simulink model "ftc_biodiesel"  (R2026b)
settings: Solver=ode15s  StopTime=120  MaxStep=0.25  RelTol=1e-7  AbsTol=1e-9
InitFcn:
  | ftc_supervisor('init', sup_cfg);
values from neighbouring files (symbols this model uses):
  P = rmfield(P, 'names')    [build_ftc_sim.m]    (also in ftc_check.m = ftc_params(); ftc_supervisor.m = S.P)
undefined symbols (not defined in the file or in its folder): ctrl_mode, t_f
libraries: slpidlib x1
settings Model: Creator=Joseph  LastModifiedBy=Joseph

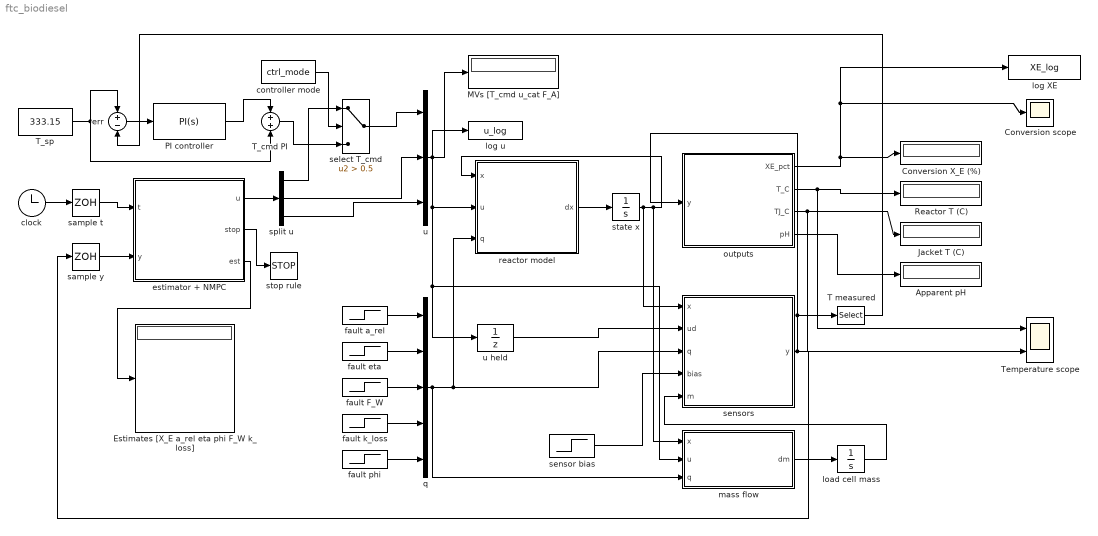
== system ftc_biodiesel ==
  Apparent pH : Display
  Conversion X_E (%) : Display
  Conversion scope : Scope
  Estimates [X_E a_rel eta phi F_W k_loss] : Display
  Jacket T (C) : Display
  MVs [T_cmd u_cat F_A] : Display
  PI controller : slpidlib/PID Controller  Controller=PI  Form=Parallel  TimeDomain=Continuous-time  UseExternalTs=off  SampleTime=-1  IntegratorMethod=Forward Euler  FilterMethod=Forward Euler  ControllerParametersSource=internal  P=6  I=6/8  UseKiTs=off  D=0  UseExternalDerivativeSource=off  N=100  UseFilter=on  TunerSelectOption=Transfer Function Based (PID Tuner App)  InitialConditionSource=internal  InitialConditionForIntegrator=0  InitialConditionForFilter=0  DifferentiatorICPrevScaledInput=0  ExternalReset=none  TrackingMode=off  Kt=1  LimitOutput=on  SatLimitsSource=internal  UpperSaturationLimit=353.15-333.15  LowerSaturationLimit=298.15-333.15  LinearizeAsGain=on  AntiWindupMode=back-calculation  Kb=1/8  LimitIntegrator=off  UpperIntegratorSaturationLimit=inf  LowerIntegratorSaturationLimit=-inf  POutMin=[]  POutMax=[]  IOutMin=[]  IOutMax=[]  DOutMin=[]  DOutMax=[]  NOutMin=[]  NOutMax=[]  SumOutMin=[]  SumOutMax=[]  SaturationOutMin=[]  SaturationOutMax=[]  PParamMin=[]  PParamMax=[]  IParamMin=[]  IParamMax=[]  DParamMin=[]  DParamMax=[]  NParamMin=[]  NParamMax=[]  KbParamMin=[]  KbParamMax=[]  KtParamMin=[]  KtParamMax=[]  KbOutMin=[]  KbOutMax=[]  KtOutMin=[]  KtOutMax=[]  IntegratorOutMin=[]  IntegratorOutMax=[]  FilterOutMin=[]  FilterOutMax=[]  SumI1OutMin=[]  SumI1OutMax=[]  SumI2OutMin=[]  SumI2OutMax=[]  SumI3OutMin=[]  SumI3OutMax=[]  SumI4OutMin=[]  SumI4OutMax=[]  SumDOutMin=[]  SumDOutMax=[]  DifferentiatorOutMin=[]  DifferentiatorOutMax=[]  FilterDiffOutCoefMin=[]  FilterDiffOutCoefMax=[]  ReciprocalOutMin=[]  ReciprocalOutMax=[]  SumDenOutMin=[]  SumDenOutMax=[]  SumNumOutMin=[]  SumNumOutMax=[]  DivideOutMin=[]  DivideOutMax=[]  UdiffTsProdOutMin=[]  UdiffTsProdOutMax=[]  NTsProdOutMin=[]  NTsProdOutMax=[]  UintegralTsProdOutMin=[]  UintegralTsProdOutMax=[]  UngainTsProdOutMin=[]  UngainTsProdOutMax=[]  ClampingZeroOutDataTypeStr=Inherit: Inherit via back propagation  ClampingZeroOutMin=[]  ClampingZeroOutMax=[]  FilterDenConstantOutDataTypeStr=Inherit: Inherit via back propagation  FilterDenConstantOutMin=[]  FilterDenConstantOutMax=[]  PCopyOutDataTypeStr=Inherit: Inherit via back propagation  PCopyOutMin=[]  PCopyOutMax=[]  NCopyOutDataTypeStr=Inherit: Inherit via back propagation  NCopyOutMin=[]  NCopyOutMax=[]  IntegratorContinuousStateAttributes=''  IntegratorStateMustResolveToSignalObject=off  IntegratorRTWStateStorageClass=Auto  FilterContinuousStateAttributes=''  FilterStateMustResolveToSignalObject=off  FilterRTWStateStorageClass=Auto  ParallelPVariant=InternalParameters  IdealPVariant=Disabled  IVariant=InternalParameters  DVariant=Disabled  IntegratorVariant=Continuous  SatVariant=Enabled  AWVariant=BackCalculation  PCopyVariant=Disabled  TRVariant=Disabled  FdbkBlocksVariant=Forward  IdealPFdbkVariant=Disabled  SatFdbkVariant=Disabled  DerivativeFilterVariant=Disabled  NVariant=Disabled  NCopyVariant=Disabled_SignalSpec  FilterICVariant=Disabled  IntegratorICVariant=InternalICs  ExternalResetVariant=Disabled  TRSumVariant=Passthrough  SumFdbkVariant=Disabled  SumVariant=Sum_PI  TsampFilterVariant=InternalTs  TsampNgainVariant=Passthrough  TsampIntegralVariant=Disabled_SignalSpec  ExternalSaturationOutDataTypeStr=Inherit: Same as second input  DerivativeSourceVariant=Disabled  PreIntVariant=InternalPreInt
  Reactor T (C) : Display
  T measured : Selector  InputPortWidth=9  IndexOptions=Index vector (dialog)  Indices=1  OutputSizes=1
  T_cmd PI : Sum
  T_sp : Constant  Value=333.15
  Temperature scope : Scope  NumInputPorts=2
  clock : Clock
  controller mode : Constant  Value=ctrl_mode
  err : Sum  Inputs=+-
  estimator + NMPC : MATLAB Function  TreatAsAtomicUnit=on
  fault F_W : Step  Time=t_f  FinalValue=FW_f  SampleTime=0
  fault a_rel : Step  Time=t_f  InitialValue=1  FinalValue=a_f  SampleTime=0
  fault eta : Step  Time=t_f  InitialValue=1  FinalValue=eta_f  SampleTime=0
  fault k_loss : Step  Time=t_f  FinalValue=kl_f  SampleTime=0
  fault phi : Step  Time=t_f  InitialValue=1  FinalValue=phi_f  SampleTime=0
  load cell mass : Integrator
  log XE : ToWorkspace  VariableName=XE_log  SaveFormat=Timeseries  SampleTime=-1
  log u : ToWorkspace  VariableName=u_log  SaveFormat=Timeseries  SampleTime=-1
  mass flow : MATLAB Function  TreatAsAtomicUnit=on
  outputs : MATLAB Function  TreatAsAtomicUnit=on
  q : Mux  Inputs=5
  reactor model : MATLAB Function  TreatAsAtomicUnit=on
  sample t : ZeroOrderHold  SampleTime=0.25
  sample y : ZeroOrderHold  SampleTime=0.25
  select T_cmd : Switch  Criteria=u2 > Threshold  Threshold=0.5  SaturateOnIntegerOverflow=off  InputSameDT=off
  sensor bias : Step  Time=t_f  FinalValue=bias_f  SampleTime=0
  sensors : MATLAB Function  TreatAsAtomicUnit=on
  split u : Demux  Outputs=3
  state x : Integrator  InitialCondition=P.x0
  stop rule : Stop
  u : Mux  Inputs=3
  u held : UnitDelay  InitialCondition=[P.x0(13); 0; 0]  SampleTime=0.25
  wires:
  T_sp/1 -> err/1, T_cmd PI/2
  err/1 -> PI controller/1
  PI controller/1 -> T_cmd PI/1
  clock/1 -> sample t/1
  sample t/1 -> estimator + NMPC/1(t)
  sample y/1 -> estimator + NMPC/2(y)
  estimator + NMPC/1(u) -> split u/1
  estimator + NMPC/2(stop) -> stop rule/1
  estimator + NMPC/3(est) -> Estimates [X_E a_rel eta phi F_W k_loss]/1
  split u/1 -> select T_cmd/1
  controller mode/1 -> select T_cmd/2
  T_cmd PI/1 -> select T_cmd/3
  select T_cmd/1 -> u/1
  split u/2 -> u/2
  split u/3 -> u/3
  u/1 -> mass flow/2(u), u held/1, reactor model/2(u), MVs [T_cmd u_cat F_A]/1, log u/1
  fault a_rel/1 -> q/1
  fault eta/1 -> q/2
  fault F_W/1 -> q/3
  fault k_loss/1 -> q/4
  fault phi/1 -> q/5
  q/1 -> reactor model/3(q), sensors/3(q), mass flow/3(q)
  reactor model/1(dx) -> state x/1
  state x/1 -> reactor model/1(x), mass flow/1(x), sensors/1(x)
  u held/1 -> sensors/2(ud)
  sensor bias/1 -> sensors/4(bias)
  load cell mass/1 -> sensors/5(m)
  mass flow/1(dm) -> load cell mass/1
  sensors/1(y) -> outputs/1(y), T measured/1, sample y/1
  T measured/1 -> err/2
  outputs/1(XE_pct) -> log XE/1, Conversion scope/1, Conversion X_E (%)/1
  outputs/2(T_C) -> Reactor T (C)/1, Temperature scope/1
  outputs/3(TJ_C) -> Jacket T (C)/1, Temperature scope/2
  outputs/4(pH) -> Apparent pH/1

== matlab function ftc_biodiesel/reactor model ==
  data: x input size=14; u input size=3; dx output size=14; q input size=5; P parameter
function dx = f(x, u, q, P)
% plant right-hand side (ftc_rhs.m)
dx = ftc_rhs(x, u, q, P);

== matlab function ftc_biodiesel/estimator + NMPC ==
  data: t input; u output; y input size=9; stop output; est output
function [u, stop, est] = f(t, y)
% causal GRU estimator and NMPC every 5 min (ftc_supervisor.m)
coder.extrinsic('ftc_supervisor');
u = zeros(3,1); stop = 0; est = zeros(6,1);
[u, stop, est] = ftc_supervisor(t, y);

== matlab function ftc_biodiesel/sensors ==
  data: x input size=14; y output size=9; ud input size=3; q input size=5; bias input; m input; P parameter
function y = f(x, ud, q, bias, m, P)
% true measured quantities (noise is added in the supervisor); ud = inputs of the last 0.25 min
Tc = min(max(ud(1), 298.15), 353.15);
Tin = x(14) + q(5) * (Tc - x(14));
Vbp = (x(5) * 32.042/0.791 + x(4) * 292/0.875) / 1000;
CB = (1/138.205) / (6*100/870*32.042/0.791/1000);
pH = 12 + log10(max(x(7) + x(11), 1e-12) / Vbp / CB);
y = [x(13) + bias; x(14); Tin; Tc; q(2); pH; P.m0 + m; x(4) / (3*P.x0(1)); x(13)];

== matlab function ftc_biodiesel/mass flow ==
  data: x input size=14; u input size=3; dm output; q input size=5
function dm = f(x, u, q)
% load-cell mass change, kg/min: methanol make-up minus loss, water ingress, catalyst top-up
dm = (u(3) - q(4)*max(x(5),0)) * 32.042/1000 + q(3) * 18.015/1000 + u(2) * 138.205/1000;

== matlab function ftc_biodiesel/outputs ==
  data: y input size=9; XE_pct output; T_C output; TJ_C output; pH output
function [XE_pct, T_C, TJ_C, pH] = f(y)
XE_pct = 100 * y(8);  T_C = y(9) - 273.15;  TJ_C = y(2) - 273.15;  pH = y(6);
